simulink model "BEV_Thermal_Management"  (R2025a)
settings: Solver=ode23t  StartTime=0  StopTime=765  MaxStep=5  RelTol=1e-3  AbsTol=1e-3
model workspace: external: MATLAB File BEV_Thermal_Management_param.m (data not in the file)
undefined symbols (not defined in the file): Battery, bulb, cabin_doors_conductivity, cabin_duct_area, cabin_glass_conductivity, cabin_roof_conductivity, cabin_T_init, chiller_area_primary, chiller_N_baffles, chiller_N_tubes, chiller_tube_D, chiller_tube_L, chiller_wall_conductivity, chiller_wall_thickness, compressor_rpm_LUT, condenser_air_area_flow, condenser_air_area_primary, condenser_W, condenser_wall_conductivity, condenser_wall_thickness, coolant_channel_D, coolant_pipe_area, coolant_pipe_D, coolant_T_init, coolant_tank_area, coolant_tank_volume, coolant_valve_D_ratio_max, coolant_valve_D_ratio_min, coolant_valve_displacement, coolant_valve_S_max, cycle, DCDC, Edrive, evaporator_air_area_flow, evaporator_air_area_primary, evaporator_W, evaporator_wall_conductivity, evaporator_wall_thickness, heater_max_power, ModuleType1, outlet, ptc_max_power, pump_speed_max, radiationReflectionShields, radiator_air_area_flow, radiator_air_area_primary, radiator_W, radiator_wall_conductivity, radiator_wall_thickness, refrigerant_alpha_init, refrigerant_pipe_D, transRatio
libraries: fl_lib x264, nesl_utility x91, SimscapeFluids_lib x22, sdl_lib x13, ee_lib x9, nesl_utility_internal x4, slpidlib x3, BatteryProtection x3, batt_lib x2, BatteryCurrentManagement x1, autolibsharedcommon x1, simulink x1
(part 4 of 9)

== system BEV_Thermal_Management/Evaporator ==
  note: The evaporator is a rectangular tube-and-fin type heat exchanger that lets the refrigerant absorb heat from the air. It also dehumidifies the air when the air is humid.
  Evaporator : SimscapeFluids_lib/Heat Exchangers/Two-Phase Fluid - Moist Air/Condenser Evaporator (2P-MA)  flow_arrangement=fluids.heat_exchangers.enum.FlowArrangement2PMA.Cross  cross_flow_arrangement=fluids.heat_exchangers.enum.CrossFlowArrangement2PMA.UnmixedUnmixed  R_wall=evaporator_wall_thickness / evaporator_air_area_primary / evaporator_wall_conductivity K/W  wall_thermal_mass=false  mass_wall=1 kg  cp_wall=490 J/(K*kg)  area_A1=pi * refrigerant_pipe_D^2 / 4 m^2  area_B1=pi * refrigerant_pipe_D^2 / 4 m^2  area_A2=cabin_duct_area m^2  area_B2=cabin_duct_area m^2  tube_num_2P=evaporator_N_tubes  tube_length_2P=evaporator_L m  tube_cross_section_2P=fluids.heat_exchangers.enum.TubeCrossSection.Rectangular  tube_diameter_2P=0.1 m  tube_width_2P=evaporator_W m  tube_height_2P=evaporator_tube_H m  tube_inner_diameter_2P=0.05 m  tube_outer_diameter_2P=0.1 m  tube_flow_area_2P=0.01 m^2  tube_wetted_perimeter_2P=0.4 m  tube_heat_perimeter_2P=0.4 m  tube_pressure_loss_spec_2P=fluids.heat_exchangers.enum.TubePressureLossSpec2P.Haaland  tube_loss_coeff_2P=10  tube_local_pressure_loss_spec_2P=fluids.heat_exchangers.enum.LocalLossSpec.AggregateLength  tube_length_add_2P=evaporator_tube_Leq m  tube_local_loss_coefficient_2P=0.1  tube_roughness_pressure_2P=15e-6 m  tube_Re_lam_pressure_2P=2000  tube_Re_tur_pressure_2P=4000  tube_shape_factor_generic_2P=64  tube_heat_coeff_spec_2P=fluids.heat_exchangers.enum.TubeHeatCoeffSpec2P.GneilinskiCavalliniZecchin  tube_colburn_coeff_liq_2P=[.023, .8, .33]  tube_colburn_coeff_mix_2P=[.05, .8, .33]  tube_colburn_coeff_vap_2P=[.023, .8, .33]  tube_roughness_heat_2P=15e-6 m  tube_Re_lam_heat_2P=2000  tube_Re_tur_heat_2P=4000  tube_Nu_lam_generic_2P=3.66  fouling_factor_2P=0.1 m^2*K/kW  fin_area_2P=evaporator_tube_area_webs m^2  fin_efficiency_2P=0.6  energy_spec_2P=foundation.enum.energy_spec.void_fraction  p_init_2P=refrigerant_p_init MPa  T_init_2P=293.15 K  x_init_2P=0.5  alpha_init_2P=refrigerant_alpha_init  h_init_2P=1500 kJ/kg  u_init_2P=1500 kJ/kg  flow_geometry_MA=fluids.heat_exchangers.enum.FlowGeometryMA.Generic  tube_num_MA=1  tube_length_MA=5 m  tube_cross_section_MA=fluids.heat_exchangers.enum.TubeCrossSection.Circular  tube_diameter_MA=0.1 m  tube_width_MA=0.1 m  tube_height_MA=0.1 m  tube_inner_diameter_MA=0.05 m  tube_outer_diameter_MA=0.1 m  tube_flow_area_MA=0.01 m^2  tube_wetted_perimeter_MA=0.4 m  tube_heat_perimeter_MA=0.4 m  tube_pressure_loss_spec_MA=fluids.heat_exchangers.enum.TubePressureLossSpec.Haaland  tube_loss_coeff_MA=10  tube_local_pressure_loss_spec_MA=fluids.heat_exchangers.enum.LocalLossSpec.AggregateLength  tube_length_add_MA=0.1 m  tube_local_loss_coefficient_MA=0.1  tube_roughness_pressure_MA=15e-6 m  tube_Re_lam_pressure_MA=2000  tube_Re_tur_pressure_MA=4000  tube_shape_factor_generic_MA=64  tube_heat_coeff_spec_MA=fluids.heat_exchangers.enum.TubeHeatCoeffSpec.Gneilinski  tube_colburn_coeff_MA=[.023, .8, .33]  tube_roughness_heat_MA=15e-6 m  tube_Re_lam_heat_MA=2000  tube_Re_tur_heat_MA=4000  tube_Nu_lam_generic_MA=3.66  bank_arrangement_MA=fluids.heat_exchangers.enum.BankArrangement.Inline  bank_num_rows_MA=5  bank_tubes_per_row_MA=5  bank_width_MA=1 m  bank_tube_diameter_MA=0.05 m  bank_longitudinal_pitch_MA=0.15 m  bank_transverse_pitch_MA=0.15 m  bank_pressure_loss_spec_MA=fluids.heat_exchangers.enum.BankPressureLossSpec.Martin  bank_euler_MA=10  bank_heat_coeff_spec_MA=fluids.heat_exchangers.enum.BankHeatCoeffSpec.Martin  bank_colburn_coeff_MA=[.27, .63, .36]  generic_flow_area_MA=evaporator_air_area_flow m^2  generic_heat_area_MA=evaporator_air_area_primary m^2  generic_volume_MA=evaporator_air_area_flow * evaporator_W m^3  generic_loss_coeff_MA=10  generic_colburn_coeff_MA=[0.27, 0.63, 0.36]  fouling_factor_MA=0.1 m^2*K/kW  fin_area_MA=evaporator_air_area_fins m^2  fin_efficiency_MA=0.7  p_init_MA=cabin_p_init MPa  T_init_MA=cabin_T_init K  humidity_spec_MA=foundation.enum.HumiditySpec.RelativeHumidity  RH_init_MA=cabin_RH_init  x_w_init_MA=0.01  y_w_init_MA=0.01  HR_init_MA=0.01  Tw_init_MA=287 K  trace_gas_spec_MA=foundation.enum.trace_gas_spec.mole_fraction  x_g_init_MA=0.001  y_g_init_MA=cabin_CO2_init  r_d_init_MA=0  RH_ws_MA=1  time_constant_cond_MA=1e-3 s  time_constant_evap_MA=1e-3 s  fraction_entrained_MA=1
      settings: InternalSimscapePortConfiguration="{\"Bottom\":[],\"Left\":[{\"id\":\"A1\",\"label\":\"A1\",\"type\":\"foundation.two_phase_fluid.two_phase_fluid\"},{\"id\":\"Z\",\"label\":\"Z\",\"type\":\"output\"},{\"id\":\"B1\",\"label\":\"B1\",\"type\":\"foundation.two_phase_fluid.two_phase_fluid\"}],\"Right\":[{\"id\":\"A2\",\"label\":\"A2\",\"type\":\"foundation.moist_air.moist_air\"},{\"id\":\"W\",\"label\":\"W\",\"type\":\"output\"},{\"id\":\"B2\",\"label\":\"B2\",\"type\":\"foundation.moist_air.moist_air\"}],\"Top\":[]}"
  Flow Resistance (2P) : fl_lib/Two-Phase Fluid/Elements/Flow Resistance (2P)  delta_p_nominal=1e-4 MPa  mdot_nominal=0.01 kg/s  v_nominal=0 m^3/kg  area=pi * refrigerant_pipe_D^2 / 4 m^2  laminar_fraction=1e-3
      settings: InternalSimscapePortConfiguration="{\"Bottom\":[],\"Left\":[{\"id\":\"A\",\"label\":\"A\",\"type\":\"foundation.two_phase_fluid.two_phase_fluid\"}],\"Right\":[{\"id\":\"B\",\"label\":\"B\",\"type\":\"foundation.two_phase_fluid.two_phase_fluid\"}],\"Top\":[]}"
  SR5 : Subsystem
      mask Display: disp(get_param(gcb, 'Name'))
  SR6 : Subsystem
      mask Display: disp(get_param(gcb, 'Name'))
  Simscape Bus : SimscapeBus  HierarchyStrings=bulb;outlet
  B : PMIOPort  Side=Left
  C : PMIOPort  Port=2  Side=Left
  A : PMIOPort  Port=3  Side=Right
  D : PMIOPort  Port=4  Side=Right
  connections:
  Simscape Bus/LConn1 -- Evaporator/LConn3 -- SR6/RConn1
  Evaporator/RConn3 -- C/RConn1
  Evaporator/RConn1 -- D/RConn1
  Evaporator/LConn1 -- SR5/LConn1
  Simscape Bus/RConn1 -- A/RConn1
  Simscape Bus/LConn2 -- SR5/RConn1
  Flow Resistance (2P)/LConn1 -- SR6/LConn1
  Flow Resistance (2P)/RConn1 -- B/RConn1

== system BEV_Thermal_Management/Heater ==
  note: The battery heater is modeled as a heat flow rate source and a thermal mass. It is turned on in cold weather to bring the battery temperature above 5 °C.
  Battery Heater : fl_lib/Thermal/Thermal Elements/Thermal Mass  mass_type=foundation.enum.constant_variable.constant  mass=2 kg  sp_heat=447 J/kg/K  mass_min=1e-6 kg  num_ports=foundation.enum.numPorts2.one  m_specify=off  m_priority=High  m=1 kg  m_nominal_specify=off  m_nominal_value=1  m_nominal_unit=kg  T_specify=on  T_priority=High  T=coolant_T_init K  T_nominal_specify=off  T_nominal_value=1  T_nominal_unit=K  Q_specify=off  Q_priority=None  Q=0 W  Q_nominal_specify=off  Q_nominal_value=1  Q_nominal_unit=W
  Controlled Heat Flow Rate Source : fl_lib/Thermal/Thermal Sources/Controlled Heat Flow Rate Source
  Convective Heat Transfer : fl_lib/Thermal/Thermal Elements/Convective Heat Transfer  thermal_type=foundation.enum.constant_variable.constant  area=1 m^2  heat_tr_coeff=400 W/(m^2 * K)  min_heat_tr_coeff=1e-3 W/(K*m^2)  T_specify=off  T_priority=None  T=0 K  T_nominal_specify=off  T_nominal_value=1  T_nominal_unit=K  Q_specify=off  Q_priority=None  Q=0 W  Q_nominal_specify=off  Q_nominal_value=1  Q_nominal_unit=W
  Current calculator : Subsystem
      settings: PortSchema="{\"entries\":[{\"content\":{\"sides\":[{\"content\":{\"connectorIds\":[\"LConn1\"]},\"type\":\"ConnectorPlacement.EquallySpacedRectSide\",\"uuid\":\"170b43eb-52b0-4cc5-ac2d-ab73c42b55a5\"},{\"content\":{\"side\":\"RIGHT\"},\"type\":\"ConnectorPlacement.EquallySpacedRectSide\",\"uuid\":\"0f0abf3e-a1f4-4f38-850a-d970da92bf07\"},{\"content\":{\"connectorIds\":[\"LConn2\"],\"side\":\"TOP\"},\"type\":\"ConnectorPlacement.EquallySpacedRectSide\",\"uuid\":\"064a69fa-4b9f-4495-8c21-6533099d7712\"}]},\"type\":\"ConnectorPlacement.EquallySpacedConnector\",\"uuid\":\"c1bba2b5-aebc-432d-9d95-55118ac968cd\"}],\"packageUris\":[\"http://schema.mathworks.com/mf0/Connector/R2020b\"],\"version\":\"1.0\"}"
      mask Display: disp('CSR2')
  Flow Resistance (TL) : fl_lib/Thermal Liquid/Elements/Flow Resistance (TL)  delta_p_nominal=4e-4 MPa  mdot_nominal=0.15 kg/s  area=coolant_pipe_area m^2  laminar_fraction=1e-3
  Flow Resistance (TL)1 : fl_lib/Thermal Liquid/Elements/Flow Resistance (TL)  delta_p_nominal=4e-4 MPa  mdot_nominal=0.15 kg/s  area=coolant_pipe_area m^2  laminar_fraction=1e-3
  Heater Coolant Volume : fl_lib/Thermal Liquid/Elements/Constant Volume Chamber (TL)  volume=0.001 m^3  num_ports=foundation.enum.num_ports.two  area_A=coolant_pipe_area m^2  area_B=coolant_pipe_area m^2  area_C=0.01 m^2  area_D=0.01 m^2  p_I_specify=on  p_I_priority=High  p_I=coolant_p_init MPa  p_I_nominal_specify=off  p_I_nominal_value=1  p_I_nominal_unit=MPa  T_I_specify=on  T_I_priority=High  T_I=coolant_T_init K  T_I_nominal_specify=off  T_I_nominal_value=1  T_I_nominal_unit=K  u_I_specify=off  u_I_priority=None  u_I=83.90600000000001 kJ/kg  u_I_nominal_specify=off  u_I_nominal_value=1  u_I_nominal_unit=kJ/kg  rho_I_specify=off  rho_I_priority=None  rho_I=998.21 kg/m^3  rho_I_nominal_specify=off  rho_I_nominal_value=1  rho_I_nominal_unit=kg/m^3
      settings: InternalSimscapePortConfiguration="{\"Bottom\":[],\"Left\":[{\"id\":\"A\",\"label\":\"A\",\"type\":\"foundation.thermal_liquid.thermal_liquid\"},{\"id\":\"H\",\"label\":\"H\",\"type\":\"foundation.thermal.thermal\"}],\"Right\":[{\"id\":\"B\",\"label\":\"B\",\"type\":\"foundation.thermal_liquid.thermal_liquid\"}],\"Top\":[]}"
  Max Power [W] : Gain  Gain=heater_max_power
  SC1 : Subsystem
      mask Display: disp(get_param(gcb, 'Name'))
  SC7 : Subsystem
      mask Display: disp(get_param(gcb, 'Name'))
  Simulink-PS Converter : nesl_utility/Simulink-PS Converter  PhysicalDomain=network_engine_domain  SubClassName=ps_input  LeftPortType=input  RightPortType=output  PseudoPeriodic=off  Frequencies=[]  NoiseDistribution=none  NoiseParameters=[]  Unit=W  AffineConversion=off  FilteringAndDerivatives=provide  SimscapeFilterOrder=1  InputFilterTimeConstant=0.001  UdotUserProvided=0
  Thermal Reference : fl_lib/Thermal/Thermal Elements/Thermal Reference
  Transfer Fcn : TransferFcn  Denominator=[1 1]
  B : PMIOPort  Side=Left
  A : PMIOPort  Port=2  Side=Left
  HV : PMIOPort  Port=3  Side=Right
  wires:
  Max Power [W]/1 -> Simulink-PS Converter/1
  Transfer Fcn/1 -> Max Power [W]/1
  [cmd_heater] -> Transfer Fcn/1  "cmdHeater"
  connections:
  Flow Resistance (TL)1/RConn1 -- SC1/LConn1
  Battery Heater/LConn1 -- Controlled Heat Flow Rate Source/LConn1 -- Convective Heat Transfer/LConn1
  Simulink-PS Converter/RConn1 -- Current calculator/LConn2 -- Controlled Heat Flow Rate Source/RConn1
  Thermal Reference/LConn1 -- Controlled Heat Flow Rate Source/RConn2
  Flow Resistance (TL)/RConn1 -- Heater Coolant Volume/LConn1
  SC7/LConn1 -- A/RConn1
  Flow Resistance (TL)1/LConn1 -- Heater Coolant Volume/RConn1
  Convective Heat Transfer/RConn1 -- Heater Coolant Volume/LConn2
  HV/RConn1 -- Current calculator/LConn1
  SC7/RConn1 -- Flow Resistance (TL)/LConn1
  SC1/RConn1 -- B/RConn1

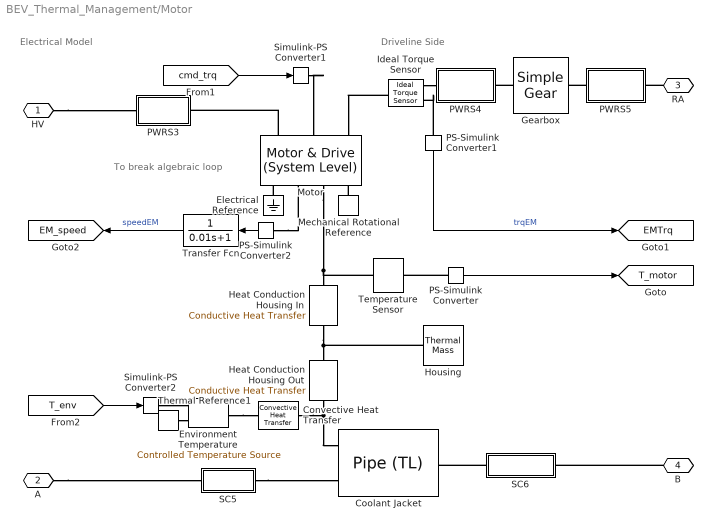
== system BEV_Thermal_Management/Motor ==
  note: Driveline Side
  note: Electrical Model
  note: To break algebraic loop
  Convective Heat Transfer : fl_lib/Thermal/Thermal Elements/Convective Heat Transfer  thermal_type=foundation.enum.constant_variable.constant  area=Edrive.diameter*pi*Edrive.length m^2  heat_tr_coeff=5 W/(K*m^2)  min_heat_tr_coeff=1e-3 W/(K*m^2)  T_specify=off  T_priority=None  T=0 K  T_nominal_specify=off  T_nominal_value=1  T_nominal_unit=K  Q_specify=off  Q_priority=None  Q=0 W  Q_nominal_specify=off  Q_nominal_value=1  Q_nominal_unit=W
  Coolant Jacket : SimscapeFluids_lib/Thermal Liquid/Pipes & Fittings/Pipe (TL)  dynamic_compressibility=simscape.enum.onoff.on  inertia=simscape.enum.onoff.off  num_segments=1  pipe_length=0.4 m  cross_section_geometry=fluids.thermal_liquid.pipes_fittings.enum.CrossSectionGeometry.Custom  pipe_diameter=0.1 m  pipe_inner_diameter=0.05 m  pipe_outer_diameter=0.1 m  pipe_width=0.1 m  pipe_height=0.1 m  pipe_major_axis=0.1 m  pipe_minor_axis=0.05 m  pipe_side=0.1 m  pipe_angle=30 deg  area=4*pi * coolant_channel_D^2 / 4 m^2  Dh=coolant_channel_D m  elevation_spec=foundation.enum.constant_variable.constant  elevation_gain=0 m  gravity_spec=foundation.enum.constant_variable.constant  g=9.81 m/s^2  pressure_loss_spec=fluids.thermal_liquid.pipes_fittings.enum.PressureLossSpec.Haaland  local_pressure_loss_spec=fluids.thermal_liquid.pipes_fittings.enum.LocalLossSpec.AggregateLength  length_add=20 * coolant_channel_D * 4 m  loss_coefficient=0.1  roughness_spec=fluids.thermal_liquid.pipes_fittings.enum.RoughnessSpec.Custom  roughness=1.5e-5 m  Re_friction_TLU=[ 400 1000 1.5e+3 3e+3 4e+3 6e+3 1e+4 2e+4 4e+4 6e+4 1e+5 1e+8 ]  friction_factor_TLU=[ 0.264 0.112 0.07099999999999999 0.0417 0.0387 0.0268 0.025 0.0232 0.0226 0.022 0.0214 0.0214 ]  Re_lam=100  Re_tur=500  shape_factor=64  mdot_nominal=[ 0.1 1 ] kg/s  p_diff_nominal=[ 0.001 0.01 ] MPa  mdot_threshold=1e-6 kg/s  wall_spec=fluids.thermal_liquid.pipes_fittings.enum.wall_spec.rigid  vol_expansion_spec=fluids.thermal_liquid.pipes_fittings.enum.VolumeExpansionSpec.Diameter  area_pressure_gain=1e-6 m^2/MPa  static_pressure_TLU=[.1, 1] MPa  area_pressure_gain_TLU=[1e-05, 1.1e-05] m^2  material_behavior_spec=fluids.thermal_liquid.pipes_fittings.enum.PipeMaterialBehavior.Linear  diameter_pressure_gain=1.2e-6 m/MPa  wall_thickness=0.05 m  elastic_modulus=69 GPa  stress_TLU=[276, 310] MPa  strain_TLU=[.004, .02]  stress_assert_action=simscape.enum.assert.action.none  stress_max=400 MPa  poisson_ratio=0.33  wall_time_constant=0.01 s  thermal_expansion=false  alpha_L_wall=24 um/(deltaK*m)  thermal_expansion_Tref=293.15 K  heat_transfer_spec=fluids.thermal_liquid.pipes_fittings.enum.HeatTransferSpec.DittusBoelter  mdot_nominal_heat=[ 0.1 1 ] kg/s  T_in_nominal=[ 293.15 293.15 ] K  T_out_nominal=[ 300 300 ] K  p_in_nominal_heat=[ 0.101325 0.101325 ] MPa  T_wall_nominal=[ 303.15 303.15 ] K  a_coeff=0.3  b_Re_power=0.8  c_Pr_power=0.33  Nu_lam=3.66  Re_Colburn_TLU=[ 100 150 1000 ]  Colburn_factor_TLU=[ 0.019 0.013 0.002 ]  Re_Nu_TLU=[ 100 150 1000 ]  Pr_Nu_TLU=[ 1 10 ]  Nu_TLU=[ 3.72 4.21; 3.75 4.44; 4.21 7.15 ]  p0_vec=coolant_p_init MPa  T0_vec=coolant_T_init K  mdot0=0.1 kg/s  p_nominal=0.101325 MPa  T_nominal=293.15 K
  Electrical Reference : fl_lib/Electrical/Electrical Elements/Electrical Reference
  Environment Temperature : fl_lib/Thermal/Thermal Sources/Controlled Temperature Source
  Gearbox : sdl_lib/Gears/Simple Gear  ratio=transRatio  rotation_direction=sdl.enum.shaftOutputDirection.same  friction_model=sdl.enum.gear_efficiencies_load.constant  T_noload=0.1 N*m  T_nom=5 N*m  efficiency_nom=0.8  efficiency=Edrive.gearboxEff  temperature_TLU=[280, 300, 320] K  load_TLU=[1, 5, 10] N*m  efficiency_TLU=[.95, .9, .85]  efficiency_TLU2=[.85, .8, .75; .95, .9, .85; .85, .8, .7]  w_thr=0.01 rad/s  pwr_thr=0.001 W  enable_backlash=false  hardstop_model=simscape.enum.hardstop.smooth  backlash_distance=1e-3 mm  r_base=0.1 m  transition=1e-4 mm  backlash_stiffness=1e6 N/m  backlash_damping=1e3 N*s/m  coeff_rest=0.7  v_tol=0.001 m/s  f_tol=0.001 N  mu_visc=[0, 0] N*m*s/rad  thermal_mass=50 J/K  temperature_specify=off  temperature_priority=High  temperature=300 K  temperature_nominal_specify=off  temperature_nominal_value=1  temperature_nominal_unit=K  x_backlash_specify=off  x_backlash_priority=None  x_backlash=0 mm  x_backlash_nominal_specify=off  x_backlash_nominal_value=1  x_backlash_nominal_unit=mm  f_hardstop_specify=off  f_hardstop_priority=None  f_hardstop=0 N  f_hardstop_nominal_specify=off  f_hardstop_nominal_value=1  f_hardstop_nominal_unit=N  v_backlash_specify=off  v_backlash_priority=None  v_backlash=0 m/s  v_backlash_nominal_specify=off  v_backlash_nominal_value=1  v_backlash_nominal_unit=m/s
  Heat Conduction Housing In : fl_lib/Thermal/Thermal Elements/Conductive Heat Transfer  thermal_type=foundation.enum.ConstantVariableTabulated.Constant  wall_geometry=foundation.enum.ConductionWallGeometry.Cylindrical  area=1e-4 m^2  thickness=0.1 m  d_in=Edrive.diameter-0.005 m  d_out=Edrive.diameter m  L=Edrive.length m  th_cond_min=10 W/(K*m)  th_cond=230 W/(K*m)  th_cond_TLU=[413, 401, 392, 383, 371, 357, 342] W/(K*m)  temp_TLU=[200, 273, 400, 600, 800, 1000, 1200] K  T_specify=off  T_priority=None  T=0 K  T_nominal_specify=off  T_nominal_value=1  T_nominal_unit=K  Q_specify=off  Q_priority=None  Q=0 W  Q_nominal_specify=off  Q_nominal_value=1  Q_nominal_unit=W
  Heat Conduction Housing Out : fl_lib/Thermal/Thermal Elements/Conductive Heat Transfer  thermal_type=foundation.enum.ConstantVariableTabulated.Constant  wall_geometry=foundation.enum.ConductionWallGeometry.Cylindrical  area=1e-4 m^2  thickness=0.1 m  d_in=Edrive.diameter-0.005 m  d_out=Edrive.diameter m  L=Edrive.length m  th_cond_min=10 W/(K*m)  th_cond=230 W/(K*m)  th_cond_TLU=[413, 401, 392, 383, 371, 357, 342] W/(K*m)  temp_TLU=[200, 273, 400, 600, 800, 1000, 1200] K  T_specify=off  T_priority=None  T=0 K  T_nominal_specify=off  T_nominal_value=1  T_nominal_unit=K  Q_specify=off  Q_priority=None  Q=0 W  Q_nominal_specify=off  Q_nominal_value=1  Q_nominal_unit=W
  Housing : fl_lib/Thermal/Thermal Elements/Thermal Mass  mass_type=foundation.enum.constant_variable.constant  mass=10 kg  sp_heat=900 J/(K*kg)  mass_min=1e-6 kg  num_ports=foundation.enum.numPorts2.one  m_specify=off  m_priority=High  m=1 kg  m_nominal_specify=off  m_nominal_value=1  m_nominal_unit=kg  T_specify=on  T_priority=High  T=coolant_T_init K  T_nominal_specify=off  T_nominal_value=1  T_nominal_unit=K  Q_specify=off  Q_priority=None  Q=0 W  Q_nominal_specify=off  Q_nominal_value=1  Q_nominal_unit=W
  Ideal Torque Sensor : fl_lib/Mechanical/Mechanical Sensors/Ideal Torque Sensor
  Mechanical Rotational Reference : fl_lib/Mechanical/Rotational Elements/Mechanical Rotational Reference
  Motor : ee_lib/Electromechanical/Motor & Drive (System Level)  torque_speed_param=ee.enum.electromech.envelope.torque_power  overtorque_param=ee.enum.electromech.overtorque.no  T_t=[.09, .08, .07, 0] N*m  T_t_intermittent=[.36, .32, .28, 0] N*m  T_t_2D=[.09, .09, .09; .08, .08, .08; .07, .07, .07; 0, 0, 0] N*m  T_t_intermittent_2D=[.36, .36, .36; .32, .32, .32; .28, .28, .28; 0, 0, 0] N*m  w_t=[0, 3750, 7500, 8000] rpm  vdc_t=[6, 12, 24] V  torque_max="Edrive.max_torque  N*m"  power_max=Edrive.max_power W  torque_max_intermittent=0.4 N*m  power_max_intermittent=120 W  time_overtorque=30 s  time_recover=60 s  Tc=Edrive.Tctc s  EnableSwitch=false  losses_param=2  eff=100  w_eff=3750 rpm  T_eff=0.08 N*m  Piron=0 W  Pbase=0 W  w_eff_vec=Edrive.loss_maps.spMat rpm  T_eff_vec=Edrive.loss_maps.tqMat N*m  v_eff_vec=[100, 250, 400] V  losses_mat=Edrive.loss_maps.lossMat W  efficiency_mat=[95, 95, 95, 95; 95, 95, 95, 95; 95, 95, 95, 95; 95, 95, 95, 95; 95, 95, 95, 95]  losses_mat_3D=ones(5, 4, 3) W  efficiency_mat_3D=95 * ones(5, 4, 3)  Res=0 Ohm  J=5e-6 kg*m^2  lam=0*1e-5 N*m*s/rad  speed0=0 rad/s  faulted_specify=off  faulted_priority=None  faulted=0  faulted_nominal_specify=off  faulted_nominal_value=1  faulted_nominal_unit=1  isSwitchedOff_specify=off  isSwitchedOff_priority=None  isSwitchedOff=0  isSwitchedOff_nominal_specify=off  isSwitchedOff_nominal_value=1  isSwitchedOff_nominal_unit=1  torqueLimitContinuous_specify=off  torqueLimitContinuous_priority=None  torqueLimitContinuous=0 N*m  torqueLimitContinuous_nominal_specify=off  torqueLimitContinuous_nominal_value=1  torqueLimitContinuous_nominal_unit=N*m  alpha=3.93e-3 1/K  Tmeas=30 degC  Tmeas2=31 degC  losses_mat_T2=Edrive.loss_maps.lossMat W  efficiency_mat_T2=[95, 95, 95, 95; 95, 95, 95, 95; 95, 95, 95, 95; 95, 95, 95, 95; 95, 95, 95, 95]  losses_mat_3D_T2=ones(5, 4, 3) W  efficiency_mat_3D_T2=95 * ones(5, 4, 3)  thermal_mass=10000 J/K  initial_temperature=coolant_T_init K
      settings: InternalSimscapePortConfiguration="{\"Bottom\":[],\"Left\":[{\"id\":\"Vp\",\"label\":\"+\",\"type\":\"foundation.electrical.electrical\"},{\"id\":\"Tr\",\"label\":\"Tr\",\"type\":\"input\"},{\"id\":\"R\",\"label\":\"R\",\"type\":\"foundation.mechanical.rotational.rotational\"}],\"Right\":[{\"id\":\"Vm\",\"label\":\"-\",\"type\":\"foundation.electrical.electrical\"},{\"id\":\"Omega\",\"label\":\"w\",\"type\":\"output\"},{\"id\":\"H\",\"label\":\"H\",\"type\":\"foundation.thermal.thermal\"},{\"id\":\"C\",\"label\":\"C\",\"type\":\"foundation.mechanical.rotational.rotational\"}],\"Top\":[]}"
  PS-Simulink Converter : nesl_utility/PS-Simulink Converter  PhysicalDomain=network_engine_domain  SubClassName=ps_output  LeftPortType=input  RightPortType=output  PseudoPeriodic=off  Frequencies=[]  VectorFormat=1-D array  Unit=degC  AffineConversion=on
  PS-Simulink Converter1 : nesl_utility/PS-Simulink Converter  PhysicalDomain=network_engine_domain  SubClassName=ps_output  LeftPortType=input  RightPortType=output  PseudoPeriodic=off  Frequencies=[]  VectorFormat=inherit  Unit=N*m  AffineConversion=off
  PS-Simulink Converter2 : nesl_utility/PS-Simulink Converter  PhysicalDomain=network_engine_domain  SubClassName=ps_output  LeftPortType=input  RightPortType=output  PseudoPeriodic=off  Frequencies=[]  VectorFormat=inherit  Unit=rad/s  AffineConversion=off
  PWRS3 : Subsystem
      mask Display: disp(get_param(gcb,'Name'));
  PWRS4 : Subsystem
      mask Display: disp(get_param(gcb,'Name'));
  PWRS5 : Subsystem
      mask Display: disp(get_param(gcb,'Name'));
  SC5 : Subsystem
      mask Display: disp(get_param(gcb, 'Name'))
  SC6 : Subsystem
      mask Display: disp(get_param(gcb, 'Name'))
  Simulink-PS Converter1 : nesl_utility/Simulink-PS Converter  PhysicalDomain=network_engine_domain  SubClassName=ps_input  LeftPortType=input  RightPortType=output  PseudoPeriodic=off  Frequencies=[]  NoiseDistribution=none  NoiseParameters=[]  Unit=N*m  AffineConversion=off  FilteringAndDerivatives=provide  SimscapeFilterOrder=1  InputFilterTimeConstant=0.001  UdotUserProvided=0
  Simulink-PS Converter2 : nesl_utility/Simulink-PS Converter  PhysicalDomain=network_engine_domain  SubClassName=ps_input  LeftPortType=input  RightPortType=output  PseudoPeriodic=off  Frequencies=[]  NoiseDistribution=none  NoiseParameters=[]  Unit=degC  AffineConversion=on  FilteringAndDerivatives=provide  SimscapeFilterOrder=1  InputFilterTimeConstant=0.001  UdotUserProvided=0
  Temperature Sensor : fl_lib/Thermal/Thermal Sensors/Temperature Sensor  temperature_measure=foundation.enum.MeasurementReference.absolute
      settings: InternalSimscapePortConfiguration="{\"Bottom\":[],\"Left\":[{\"id\":\"A\",\"label\":\"A\",\"type\":\"foundation.thermal.thermal\"}],\"Right\":[{\"id\":\"T\",\"label\":\"T\",\"type\":\"output\"}],\"Top\":[]}"
  Thermal Reference1 : fl_lib/Thermal/Thermal Elements/Thermal Reference
  Transfer Fcn : TransferFcn  Denominator=[0.01 1]
  HV : PMIOPort  Side=Left
  A : PMIOPort  Port=2  Side=Left
  RA : PMIOPort  Port=3  Side=Right
  B : PMIOPort  Port=4  Side=Right
  tag scope: EMTrq=global, EM_speed=global, T_motor=global
  wires:
  PS-Simulink Converter/1 -> [T_motor]
  [cmd_trq] -> Simulink-PS Converter1/1
  PS-Simulink Converter1/1 -> [EMTrq]  "trqEM"
  PS-Simulink Converter2/1 -> Transfer Fcn/1
  Transfer Fcn/1 -> [EM_speed]  "speedEM"
  [T_env] -> Simulink-PS Converter2/1
  connections:
  Heat Conduction Housing In/RConn1 -- Heat Conduction Housing Out/LConn1 -- Housing/LConn1
  B/RConn1 -- SC6/RConn1
  A/RConn1 -- SC5/LConn1
  PS-Simulink Converter/LConn1 -- Temperature Sensor/RConn1
  SC5/RConn1 -- Coolant Jacket/LConn1
  SC6/LConn1 -- Coolant Jacket/RConn1
  Electrical Reference/LConn1 -- Motor/RConn1
  Mechanical Rotational Reference/LConn1 -- Motor/RConn4
  Simulink-PS Converter1/RConn1 -- Motor/LConn2
  RA/RConn1 -- PWRS5/RConn1
  PS-Simulink Converter1/LConn1 -- Ideal Torque Sensor/RConn2
  Ideal Torque Sensor/LConn1 -- Motor/LConn3
  Ideal Torque Sensor/RConn1 -- PWRS4/LConn1
  Gearbox/LConn1 -- PWRS4/RConn1
  PWRS5/LConn1 -- Gearbox/RConn1
  HV/RConn1 -- PWRS3/LConn1
  Motor/LConn1 -- PWRS3/RConn1
  PS-Simulink Converter2/LConn1 -- Motor/RConn2
  Motor/RConn3 -- Temperature Sensor/LConn1 -- Heat Conduction Housing In/LConn1
  Heat Conduction Housing Out/RConn1 -- Coolant Jacket/LConn2 -- Convective Heat Transfer/LConn1
  Simulink-PS Converter2/RConn1 -- Environment Temperature/RConn1
  Thermal Reference1/LConn1 -- Environment Temperature/RConn2
  Environment Temperature/LConn1 -- Convective Heat Transfer/RConn1

== system BEV_Thermal_Management/Motor Pump ==
  Controlled Current Source : fl_lib/Electrical/Electrical Sources/Controlled Current Source
  Electrical Reference : fl_lib/Electrical/Electrical Elements/Electrical Reference
  Electrical Reference1 : fl_lib/Electrical/Electrical Elements/Electrical Reference
  Ideal Angular Velocity Source : fl_lib/Mechanical/Mechanical Sources/Ideal Angular Velocity Source
  Max Speed [rpm] : Gain  Gain=pump_speed_max
  Mechanical Rotational Reference : fl_lib/Mechanical/Rotational Elements/Mechanical Rotational Reference
  Motor Pump : SimscapeFluids_lib/Thermal Liquid/Pumps & Motors/Centrifugal Pump (TL)  pump_parameterization=fluids.thermal_liquid.pumps_motors.enum.CentrifugalPumpParameterization.Nominal  capacity_ref_nominal=20 lpm  head_ref_nominal=10 m  power_ref_nominal=120 W  head_ref_max=15 m  capacity_ref_max=40 lpm  omega_ref_analytic=1000 rpm  flow_rate_1D_TLU=[16.67, 30, 40, 53.33, 66.67, 83.33] lpm  head_1D_TLU=[50, 47.5, 45, 40, 35, 25] m  power_1D_TLU=[.6, .75, .85, .93, .98, .99] kW  omega_ref_1D=3500 rpm  rho_ref_1D=998.21 kg/m^3  omega_threshold_factor=1e-2  flow_rate_2D_TLU=[16.67, 23.33, 30, 40, 53.33, 60] lpm  omega_2D_TLU=[2450, 2800, 3150, 3500] rpm  head_2D_TLU=[25, 32.7, 42.5, 50; 24, 31.7, 41, 49; 22.7, 30.5, 39, 47.5; 20, 28, 36, 45; 15.7, 24, 32, 40; 12.5, 21, 29.5, 37.5] m  power_2D_TLU=[.28, .38, .5, .6; .31, .41, .55, .68; .33, .44, .6, .75; .36, .48, .65, .83; .38, .53, .72, .93; .39, .55, .75, .97] kW  rho_ref_2D=998.21 kg/m^3  diameter_ratio=1  mech_orientation=fluids.thermal_liquid.pumps_motors.enum.CentrifugalPumpMechOrientation.Positive  area=coolant_pipe_area m^2  operation_check=simscape.enum.assert.action.none
      settings: InternalSimscapePortConfiguration="{\"Bottom\":[],\"Left\":[{\"id\":\"A\",\"label\":\"A\",\"type\":\"foundation.thermal_liquid.thermal_liquid\"},{\"id\":\"B\",\"label\":\"B\",\"type\":\"foundation.thermal_liquid.thermal_liquid\"}],\"Right\":[{\"id\":\"R\",\"label\":\"R\",\"type\":\"foundation.mechanical.rotational.rotational\"},{\"id\":\"C\",\"label\":\"C\",\"type\":\"foundation.mechanical.rotational.rotational\"}],\"Top\":[]}"
  Power sensor : Subsystem
      settings: PortSchema="{\"entries\":[{\"content\":{\"sides\":[{\"content\":{\"connectorIds\":[\"LConn1\"]},\"type\":\"ConnectorPlacement.EquallySpacedRectSide\",\"uuid\":\"14aacb84-4d2c-4fe3-9667-966fc9affdc2\"},{\"content\":{\"connectorIds\":[\"RConn1\"],\"side\":\"RIGHT\"},\"type\":\"ConnectorPlacement.EquallySpacedRectSide\",\"uuid\":\"5f04cc75-bf75-44ff-ad13-d2b18990cf19\"},{\"content\":{\"connectorIds\":[\"LConn2\"],\"side\":\"TOP\"},\"type\":\"ConnectorPlacement.EquallySpacedRectSide\",\"uuid\":\"fdf9b4dd-6b03-4f92-a45a-c9cb867bd95a\"}]},\"type\":\"ConnectorPlacement.EquallySpacedConnector\",\"uuid\":\"3effddba-6f65-4497-8868-e18a0983ff0c\"}],\"packageUris\":[\"http://schema.mathworks.com/mf0/Connector/R2020b\"],\"version\":\"1.0\"}"
  Pump power : fl_lib/Physical Signals/Functions/PS Divide
  Simulink-PS Converter : nesl_utility/Simulink-PS Converter  PhysicalDomain=network_engine_domain  SubClassName=ps_input  LeftPortType=input  RightPortType=output  PseudoPeriodic=off  Frequencies=[]  NoiseDistribution=none  NoiseParameters=[]  Unit=rpm  AffineConversion=off  FilteringAndDerivatives=provide  SimscapeFilterOrder=1  InputFilterTimeConstant=0.001  UdotUserProvided=0
  Transfer Fcn : TransferFcn  Denominator=[5 1]
  Voltage Sensor : fl_lib/Electrical/Electrical Sensors/Voltage Sensor
  LV : PMIOPort  Side=Left
  A : PMIOPort  Port=2  Side=Left
  B : PMIOPort  Port=3  Side=Right
  wires:
  Max Speed [rpm]/1 -> Simulink-PS Converter/1
  Transfer Fcn/1 -> Max Speed [rpm]/1
  [cmd_motor_pump] -> Transfer Fcn/1
  connections:
  B/RConn1 -- Motor Pump/LConn2
  A/RConn1 -- Motor Pump/LConn1
  Motor Pump/RConn1 -- Power sensor/RConn1
  Ideal Angular Velocity Source/RConn2 -- Motor Pump/RConn2 -- Mechanical Rotational Reference/LConn1
  Simulink-PS Converter/RConn1 -- Ideal Angular Velocity Source/RConn1
  Ideal Angular Velocity Source/LConn1 -- Power sensor/LConn1
  Controlled Current Source/RConn2 -- Voltage Sensor/LConn1 -- LV/RConn1
  Electrical Reference/LConn1 -- Voltage Sensor/RConn2
  Pump power/LConn1 -- Power sensor/LConn2
  Voltage Sensor/RConn1 -- Pump power/LConn2
  Electrical Reference1/LConn1 -- Controlled Current Source/LConn1
  Pump power/RConn1 -- Controlled Current Source/RConn1

== system BEV_Thermal_Management/PTC ==
  Absolute Reference (MA) : fl_lib/Moist Air/Elements/Absolute Reference (MA)
  Controlled Heat Flow Rate Source : fl_lib/Thermal/Thermal Sources/Controlled Heat Flow Rate Source
  Convective Heat Transfer : fl_lib/Thermal/Thermal Elements/Convective Heat Transfer  thermal_type=foundation.enum.constant_variable.constant  area=1 m^2  heat_tr_coeff=200 W/(m^2 * K)  min_heat_tr_coeff=1e-3 W/(K*m^2)  T_specify=off  T_priority=None  T=0 K  T_nominal_specify=off  T_nominal_value=1  T_nominal_unit=K  Q_specify=off  Q_priority=None  Q=0 W  Q_nominal_specify=off  Q_nominal_value=1  Q_nominal_unit=W
  Current calculator : Subsystem
      settings: PortSchema="{\"entries\":[{\"content\":{\"sides\":[{\"content\":{\"connectorIds\":[\"LConn1\"]},\"type\":\"ConnectorPlacement.EquallySpacedRectSide\",\"uuid\":\"170b43eb-52b0-4cc5-ac2d-ab73c42b55a5\"},{\"content\":{\"side\":\"RIGHT\"},\"type\":\"ConnectorPlacement.EquallySpacedRectSide\",\"uuid\":\"0f0abf3e-a1f4-4f38-850a-d970da92bf07\"},{\"content\":{\"connectorIds\":[\"LConn2\"],\"side\":\"TOP\"},\"type\":\"ConnectorPlacement.EquallySpacedRectSide\",\"uuid\":\"064a69fa-4b9f-4495-8c21-6533099d7712\"}]},\"type\":\"ConnectorPlacement.EquallySpacedConnector\",\"uuid\":\"c1bba2b5-aebc-432d-9d95-55118ac968cd\"}],\"packageUris\":[\"http://schema.mathworks.com/mf0/Connector/R2020b\"],\"version\":\"1.0\"}"
      mask Display: disp('CSR1')
  Flow Resistance (MA) : fl_lib/Moist Air/Elements/Flow Resistance (MA)  delta_p_nominal=2e-4 MPa  mdot_nominal=0.15 kg/s  rho_nominal=1.2 kg/m^3  area=cabin_duct_area m^2  laminar_fraction=1e-3
  Flow Resistance (MA)1 : fl_lib/Moist Air/Elements/Flow Resistance (MA)  delta_p_nominal=2e-4 MPa  mdot_nominal=0.15 kg/s  rho_nominal=1.2 kg/m^3  area=cabin_duct_area m^2  laminar_fraction=1e-3
  Max Power [W] : Gain  Gain=ptc_max_power
  PS-Simulink Converter : nesl_utility/PS-Simulink Converter  PhysicalDomain=network_engine_domain  SubClassName=ps_output  LeftPortType=input  RightPortType=output  PseudoPeriodic=off  Frequencies=[]  VectorFormat=1-D array  Unit=degC  AffineConversion=on
  PTC Heater : fl_lib/Thermal/Thermal Elements/Thermal Mass  mass_type=foundation.enum.constant_variable.constant  mass=1.5 kg  sp_heat=447 J/kg/K  mass_min=1e-6 kg  num_ports=foundation.enum.numPorts2.one  m_specify=off  m_priority=High  m=1 kg  m_nominal_specify=off  m_nominal_value=1  m_nominal_unit=kg  T_specify=on  T_priority=High  T=cabin_T_init K  T_nominal_specify=off  T_nominal_value=1  T_nominal_unit=K  Q_specify=off  Q_priority=None  Q=0 W  Q_nominal_specify=off  Q_nominal_value=1  Q_nominal_unit=W
  PTC Air Volume : fl_lib/Moist Air/Elements/Constant Volume Chamber (MA)  volume=0.001 m^3  num_ports=foundation.enum.num_ports.two  area_A=cabin_duct_area m^2  area_B=cabin_duct_area m^2  area_C=0.01 m^2  area_D=0.01 m^2  RH_ws=1  time_constant_cond=1e-3 s  time_constant_evap=1e-3 s  fraction_entrained=1  moisture_trace_gas_source=foundation.enum.moisture_trace_gas_source.none  moisture_source_spec=foundation.enum.MoistureSourceSpec.WaterVapor  vapor_from_liquid=false  moisture_mass_flow=0 kg/s  moisture_temperature_spec=foundation.enum.temperature_spec.atmospheric  moisture_temperature=293.15 K  trace_gas_mass_flow=0 kg/s  trace_gas_temperature_spec=foundation.enum.temperature_spec.atmospheric  trace_gas_temperature=293.15 K  p_init=cabin_p_init MPa  p_init_priority=foundation.enum.Priority.High  T_init=cabin_T_init K  T_init_priority=foundation.enum.Priority.High  humidity_spec=foundation.enum.HumiditySpec.RelativeHumidity  RH_init=cabin_RH_init  RH_init_priority=foundation.enum.Priority.High  x_w_init=0  x_w_init_priority=foundation.enum.Priority.None  y_w_init=0  y_w_init_priority=foundation.enum.Priority.None  HR_init=0  HR_init_priority=foundation.enum.Priority.None  Tw_init=287 K  Tw_init_priority=foundation.enum.Priority.High  trace_gas_spec=foundation.enum.trace_gas_spec.mole_fraction  x_g_init=0  x_g_init_priority=foundation.enum.Priority.None  y_g_init=cabin_CO2_init  y_g_init_priority=foundation.enum.Priority.High  r_d_init=0  r_d_init_priority=foundation.enum.Priority.High
      settings: InternalSimscapePortConfiguration="{\"Bottom\":[],\"Left\":[{\"id\":\"A\",\"label\":\"A\",\"type\":\"foundation.moist_air.moist_air\"},{\"id\":\"B\",\"label\":\"B\",\"type\":\"foundation.moist_air.moist_air\"}],\"Right\":[{\"id\":\"W\",\"label\":\"W\",\"type\":\"output\"},{\"id\":\"F\",\"label\":\"F\",\"type\":\"output\"},{\"id\":\"H\",\"label\":\"H\",\"type\":\"foundation.thermal.thermal\"}],\"Top\":[]}"
  Pressure & Temperature Sensor (MA) : fl_lib/Moist Air/Sensors/Pressure & Temperature Sensor (MA)  reference=foundation.enum.MeasurementReference.difference  pressure=true  pressure_spec=foundation.enum.PressureMeasementSpec.Absolute  temperature=true
      settings: InternalSimscapePortConfiguration="{\"Bottom\":[{\"id\":\"T\",\"label\":\"T\",\"type\":\"output\"}],\"Left\":[{\"id\":\"A\",\"label\":\"A\",\"type\":\"foundation.moist_air.moist_air\"}],\"Right\":[{\"id\":\"B\",\"label\":\"B\",\"type\":\"foundation.moist_air.moist_air\"},{\"id\":\"P\",\"label\":\"P\",\"type\":\"output\"}],\"Top\":[]}"
  Simulink-PS Converter : nesl_utility/Simulink-PS Converter  PhysicalDomain=network_engine_domain  SubClassName=ps_input  LeftPortType=input  RightPortType=output  PseudoPeriodic=off  Frequencies=[]  NoiseDistribution=none  NoiseParameters=[]  Unit=W  AffineConversion=off  FilteringAndDerivatives=provide  SimscapeFilterOrder=1  InputFilterTimeConstant=0.001  UdotUserProvided=0
  Thermal Reference : fl_lib/Thermal/Thermal Elements/Thermal Reference
  Transfer Fcn : TransferFcn  Denominator=[1 1]
  HV : PMIOPort  Side=Left
  A : PMIOPort  Port=2  Side=Left
  B : PMIOPort  Port=3  Side=Right
  tag scope: T_ptc=global
  wires:
  Max Power [W]/1 -> Simulink-PS Converter/1
  Transfer Fcn/1 -> Max Power [W]/1
  [cmd_ptc] -> Transfer Fcn/1
  PS-Simulink Converter/1 -> [T_ptc]
  connections:
  PTC Heater/LConn1 -- Convective Heat Transfer/LConn1 -- Controlled Heat Flow Rate Source/LConn1
  Thermal Reference/LConn1 -- Controlled Heat Flow Rate Source/RConn2
  Pressure & Temperature Sensor (MA)/LConn1 -- Flow Resistance (MA)1/RConn1 -- B/RConn1
  Pressure & Temperature Sensor (MA)/RConn3 -- PS-Simulink Converter/LConn1
  Absolute Reference (MA)/LConn1 -- Pressure & Temperature Sensor (MA)/RConn1
  Convective Heat Transfer/RConn1 -- PTC Air Volume/RConn3
  Flow Resistance (MA)/RConn1 -- PTC Air Volume/LConn1
  PTC Air Volume/LConn2 -- Flow Resistance (MA)1/LConn1
  A/RConn1 -- Flow Resistance (MA)/LConn1
  Simulink-PS Converter/RConn1 -- Controlled Heat Flow Rate Source/RConn1 -- Current calculator/LConn2
  HV/RConn1 -- Current calculator/LConn1
